simulink model "comm8qamtxrxhdl"  (R2025b)
settings: Solver=FixedStepDiscrete  StartTime=0.0  StopTime=20000*qam_params.symbolPeriod  RelTol=1e-3
PreLoadFcn:
  | qam_params = comm8qamtxrxhdl_init;
InitFcn:
  | qam_params = comm8qamtxrxhdl_init;
StopFcn:
  | comm8qamtxrxhdl_analyze;
undefined symbols (not defined in the file or in its folder): Add, Shift
libraries: hdlsllib x5, dspsigops x2, dspmlti4 x2, commchan3 x1, commrflib2 x1, simulink x1, dsphdlmathfun2 x1, dsphdlsigops2 x1, simulink_need_slupdate x1, commdigbbndam3 x1, commsequence2 x1
settings Model: Creator=The MathWorks, Inc.  LastModifiedBy=Ubaid
settings SolverCC: AlgebraicLoopSolver=TrustRegion  MaxZcPerStep=1.0
settings DataIOCC: LimitDataPoints=on  SaveFormat=Array  SaveOutput=off  SaveTime=off  ReturnWorkspaceOutputs=off
settings OptimizationCC: BlockReduction=off  ConditionallyExecuteInputs=off  DefaultParameterBehavior=Inlined  ReuseModelBlockBuffer=off  LifeSpan=inf
settings DebuggingCC: AlgebraicLoopMsg=error  UnderspecifiedInitializationDetection=Classic  MergeDetectMultiDrivingBlocksExec=none  SolverPrmCheckMsg=warning  MultiTaskDSMMsg=warning  MultiTaskCondExecSysMsg=none  SingleTaskRateTransMsg=error  IntegerOverflowMsg=none  ParameterPrecisionLossMsg=none  UnconnectedInputMsg=warning  UnconnectedOutputMsg=warning  UnconnectedLineMsg=warning  AllowSymbolicDim=off  StateNameClashWarn=warning  SFUnexpectedBacktrackingDiag=warning  SFNoUnconditionalDefaultTransitionDiag=warning  SFExecutionAtInitializationDiag=none  IntegerSaturationMsg=none  ArithmeticOperatorsInVariantConditions=warning
settings HardwareCC: ProdBitPerPointer=32.0  ProdBitPerSizeT=32.0  ProdBitPerPtrDiffT=32.0  ProdLargestAtomicFloat=None  ProdIntDivRoundTo=Undefined  ProdEndianess=Unspecified  ProdWordSize=32.0  ProdHWDeviceType=ASIC/FPGA->ASIC/FPGA  ProdEqTarget=off
settings ModelReferenceCC: EnableRefExpFcnMdlSchedulingChecks=on  PropagateSignalLabelsOutOfModel=off
settings SFSimCC: SimUseLocalCustomCode=off  CustomCodeUndefinedFunction=UseInterfaceOnly
settings RTWCC: RTWUseLocalCustomCode=off  GPUComputeCapability=3.5  DLArmComputeVersion=19.05
settings CodeAppCC: StateflowObjectComments=on
settings GRTTargetCC: TargetLangStandard=C89/C90 (ANSI)
settings ConfigComp: CovMetricSettings=dw  CovSaveCumulativeToWorkspaceVar=on  CovSaveSingleToWorkspaceVar=on  CovExternalEMLEnable=off  CovSFcnEnable=off

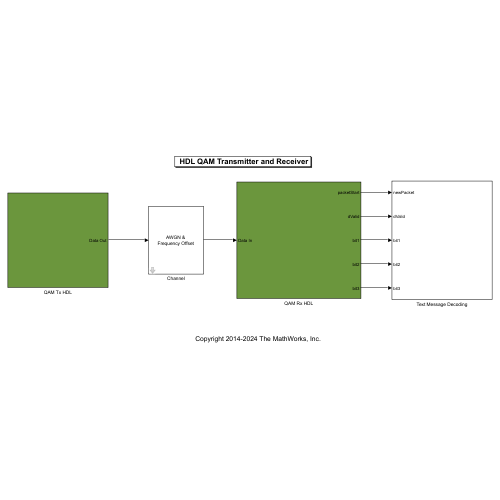
[thumbnail: Simulink's stored preview of the top-level diagram]
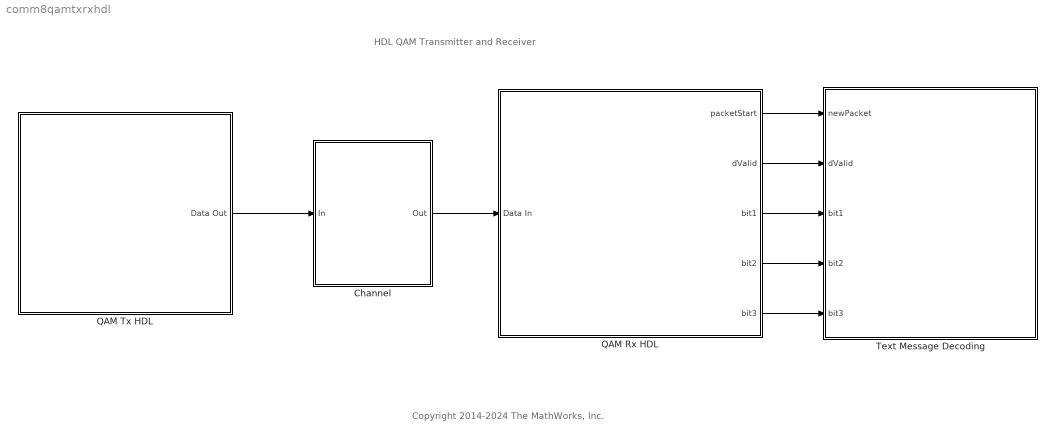
== system comm8qamtxrxhdl ==
  note: Copyright 2014-2024 The MathWorks, Inc.
  note: HDL QAM Transmitter and Receiver
  Channel : Subsystem  mask{Poff=qam_params.phaseOffset, Foff=qam_params.frequencyOffset, EbNo=qam_params.EbNo, Chan_Gain=qam_params.channelGain, Chan_Delay=qam_params.channelDelay}
      mask prompts: Poff "Phase offset (deg)"; Foff "Frequency offset (Hz)"; EbNo "Eb/No"; Chan_Gain "Channel Gain"; Chan_Delay "Channel Delay"
      mask Display: disp('AWGN &\nFrequency Offset');
  QAM Rx HDL : Subsystem
  QAM Tx HDL : Subsystem
  Text Message Decoding : Subsystem
  wires:
  QAM Rx HDL/1(packetStart) -> Text Message Decoding/1(newPacket)
  QAM Rx HDL/3(bit1) -> Text Message Decoding/3(bit1)
  QAM Rx HDL/4(bit2) -> Text Message Decoding/4(bit2)
  QAM Rx HDL/5(bit3) -> Text Message Decoding/5(bit3)
  QAM Rx HDL/2(dValid) -> Text Message Decoding/2(dValid)
  Channel/1(Out) -> QAM Rx HDL/1(Data In)
  QAM Tx HDL/1(Data Out) -> Channel/1(In)

== system comm8qamtxrxhdl/Channel ==
  In : Inport
  AWGN Channel2 : commchan3/AWGN Channel  LegacyMode=on  NoiseMethod="Signal to noise ratio  (Eb/No)"  noiseMode="Signal to noise ratio  (SNR)"  EbNo=EbNo  EsNo=15  SNR=15  BitsPerSymbol=3  SignalPower=0.11  SpecifySymbolPeriod=off  SamplesPerSymbol=1  SymbolPeriod=1/qam_params.sampleRate  VarianceSource=Parameter  Variance=1  RandomStream=Global stream  Seed=67  SimulateUsing=Code generation
  Constant : Constant  Value=Chan_Delay  SampleTime=1/qam_params.sampleRate
  Data Type Conversion1 : DataTypeConversion  OutDataTypeStr=fixdt(1,16,15)  SaturateOnIntegerOverflow=off  RndMeth=Floor
  Data Type Conversion4 : DataTypeConversion  OutDataTypeStr=double  SaturateOnIntegerOverflow=off  RndMeth=Floor
  Gain : Gain  Gain=Chan_Gain
  Phase/ Frequency Offset1 : commrflib2/Phase// Frequency Offset  phaseOffset=Poff  freqPort=off  freqOffset=Foff
  Variable Fractional Delay : dspsigops/Variable Fractional Delay  mode=OBSOLETE  modeActive=Linear  L=4  FarrowL=4  R=10  alpha=1  dmax=56*4  ic=0  noDFT=off  fallbackFIR=Clip to the minimum value necessary for centered kernel  fallbackFarrow=Clip to the minimum value necessary for centered kernel  roundingMode=Zero  overflowMode=off
  Out : Outport  VectorParamsAs1DForOutWhenUnconnected=off
  wires:
  In/1 -> Data Type Conversion4/1
  AWGN Channel2/1 -> Gain/1
  Data Type Conversion1/1 -> Out/1
  Data Type Conversion4/1 -> Phase/ Frequency Offset1/1
  Phase/ Frequency Offset1/1 -> Variable Fractional Delay/1
  Variable Fractional Delay/1 -> AWGN Channel2/1
  Constant/1 -> Variable Fractional Delay/2
  Gain/1 -> Data Type Conversion1/1

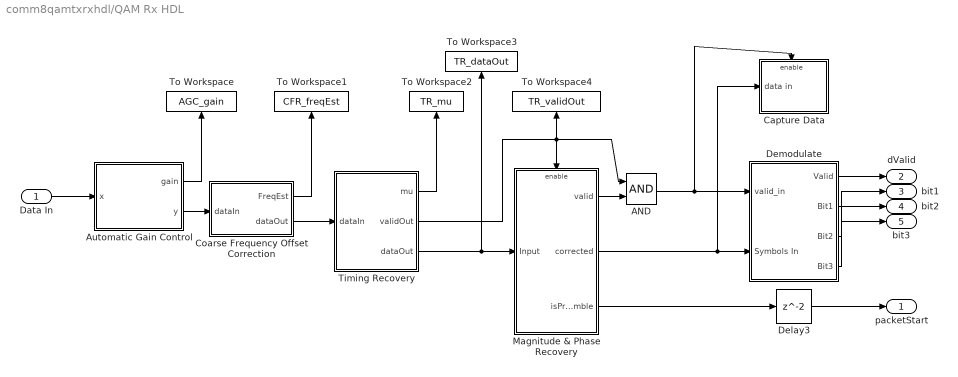
== system comm8qamtxrxhdl/QAM Rx HDL ==
  Data In : Inport
  AND : Logic  AllPortsSameDT=off  OutDataTypeStr=boolean
  Automatic Gain Control : Subsystem  mask{AGC_Ref=.23, AGC_Gain=0.001}
      mask prompts: AGC_Ref "Target Amplitude"; AGC_Gain "AGC Loop Gain"
  Capture Data : Subsystem
  Coarse Frequency Offset Correction : Subsystem
  Delay3 : Delay  InitialCondition=0
  Demodulate : Subsystem
  Magnitude & Phase Recovery : Subsystem  mask{PreAmb=qam_params.preambleRx.', threshold=1.1, LMS_Step=1/4}
      mask prompts: PreAmb "Preamble symbols"; LMS_Step "LMS step size"
  Timing Recovery : Subsystem
  To Workspace : ToWorkspace  VariableName=AGC_gain  SaveFormat=Timeseries  SampleTime=-1
  To Workspace1 : ToWorkspace  VariableName=CFR_freqEst  SaveFormat=Timeseries  SampleTime=-1
  To Workspace2 : ToWorkspace  VariableName=TR_mu  SaveFormat=Timeseries  SampleTime=-1
  To Workspace3 : ToWorkspace  VariableName=TR_dataOut  SaveFormat=Timeseries  SampleTime=-1
  To Workspace4 : ToWorkspace  VariableName=TR_validOut  SaveFormat=Timeseries  SampleTime=-1
  packetStart : Outport  VectorParamsAs1DForOutWhenUnconnected=off
  dValid : Outport  Port=2  VectorParamsAs1DForOutWhenUnconnected=off
  bit1 : Outport  Port=3  VectorParamsAs1DForOutWhenUnconnected=off
  bit2 : Outport  Port=4  VectorParamsAs1DForOutWhenUnconnected=off
  bit3 : Outport  Port=5  VectorParamsAs1DForOutWhenUnconnected=off
  wires:
  Timing Recovery/3(dataOut) -> Magnitude & Phase Recovery/1(Input), To Workspace3/1
  Demodulate/2(Bit1) -> bit1/1
  Demodulate/3(Bit2) -> bit2/1
  Demodulate/4(Bit3) -> bit3/1
  Magnitude & Phase Recovery/3(isPreamble) -> Delay3/1
  Demodulate/1(Valid) -> dValid/1
  Timing Recovery/2(validOut) -> AND/1, To Workspace4/1, Magnitude & Phase Recovery/Enable
  Data In/1 -> Automatic Gain Control/1(x)
  Automatic Gain Control/1(gain) -> To Workspace/1
  Automatic Gain Control/2(y) -> Coarse Frequency Offset Correction/1(dataIn)
  Coarse Frequency Offset Correction/2(dataOut) -> Timing Recovery/1(dataIn)
  Delay3/1 -> packetStart/1
  Magnitude & Phase Recovery/1(valid) -> AND/2
  AND/1 -> Demodulate/1(valid_in), Capture Data/Enable
  Magnitude & Phase Recovery/2(corrected) -> Demodulate/2(Symbols In), Capture Data/1(data in)
  Coarse Frequency Offset Correction/1(FreqEst) -> To Workspace1/1
  Timing Recovery/1(mu) -> To Workspace2/1

== system comm8qamtxrxhdl/QAM Tx HDL ==
  " Zero" : Constant  Value=complex(0,0)  OutDataTypeStr=fixdt(1,16,15)  SampleTime=qam_params.symbolPeriod
  Data Generation & Packetization : Subsystem
  Input Mux : MultiPortSwitch  DataPortOrder=Zero-based contiguous  Inputs=2  zeroidx=on  SaturateOnIntegerOverflow=off  InputSameDT=off
  Pipeline{1..5} (5 alike) : Delay  DelayLength=1  InitialCondition=0
  Pulse Shaping : Subsystem
  Symbol Mapping : Subsystem
  Data Out : Outport  VectorParamsAs1DForOutWhenUnconnected=off
  wires:
  Pipeline4/1 -> Input Mux/3
  Pipeline5/1 -> Data Out/1
  Pipeline1/1 -> Symbol Mapping/1(Valid In)
  Pipeline3/1 -> Input Mux/1
  " Zero"/1 -> Input Mux/2
  Data Generation & Packetization/1(Valid Out) -> Pipeline1/1
  Data Generation & Packetization/2(Raw Data) -> Pipeline2/1
  Pipeline2/1 -> Symbol Mapping/2(Integer In)
  Symbol Mapping/2(Symbol Out) -> Pipeline4/1
  Symbol Mapping/1(Valid out) -> Pipeline3/1
  Input Mux/1 -> Pulse Shaping/1(dataIn)
  Pulse Shaping/1(dataOut) -> Pipeline5/1

== system comm8qamtxrxhdl/Text Message Decoding ==
  newPacket : Inport
  dValid : Inport  Port=2
  bit1 : Inport  Port=3
  bit2 : Inport  Port=4
  bit3 : Inport  Port=5
  " " : MATLAB Function  TreatAsAtomicUnit=on
  Descramble and Print : Subsystem  TreatAsAtomicUnit=on
  wires:
  bit1/1 -> " "/3(bit1)
  bit2/1 -> " "/4(bit2)
  " "/2(framed_data) -> Descramble and Print/1(In1)
  " "/1(RxGo) -> Descramble and Print/Enable
  bit3/1 -> " "/5(bit3)
  dValid/1 -> " "/2(dValid)
  newPacket/1 -> " "/1(newPacket)

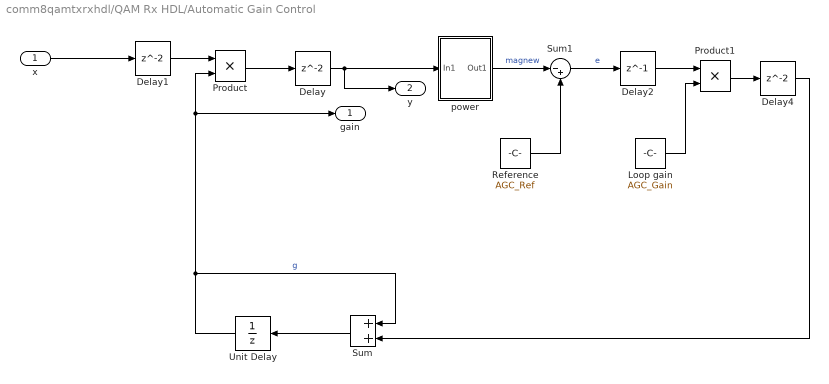
== system comm8qamtxrxhdl/QAM Rx HDL/Automatic Gain Control ==
  x : Inport
  Delay : Delay  InitialCondition=0
  Delay1 : Delay  InitialCondition=0
  Delay2 : Delay  DelayLength=1  InitialCondition=0
  Delay4 : Delay  InitialCondition=0
  Loop gain : Constant  Value=AGC_Gain  OutDataTypeStr=fixdt(1,16,15)  SampleTime=1/qam_params.sampleRate
  Product : Product  OutDataTypeStr=fixdt(1,16,15)  SaturateOnIntegerOverflow=on
  Product1 : Product  OutDataTypeStr=fixdt(1,16,15)  SaturateOnIntegerOverflow=on
  Reference : Constant  Value=AGC_Ref  OutDataTypeStr=fixdt(1,16,15)  SampleTime=1/qam_params.sampleRate
  Sum : Sum  OutDataTypeStr=Inherit: Same as accumulator  AccumDataTypeStr=fixdt(1,24,15)  SaturateOnIntegerOverflow=on
  Sum1 : Sum  Inputs=|-+  OutDataTypeStr=Inherit: Same as first input
  Unit Delay : UnitDelay  InitialCondition=.5  SampleTime=-1  HasFrameUpgradeWarning=on
  power : Subsystem
  gain : Outport  VectorParamsAs1DForOutWhenUnconnected=off
  y : Outport  Port=2  PortDimensions=1  VectorParamsAs1DForOutWhenUnconnected=off
  wires:
  Product/1 -> Delay/1
  Delay/1 -> y/1, power/1(In1)
  Sum1/1 -> Delay2/1  "e"
  Delay2/1 -> Product1/1
  Product1/1 -> Delay4/1
  Unit Delay/1 -> gain/1, Product/2, Sum/1  "g"
  Delay4/1 -> Sum/2
  x/1 -> Delay1/1
  Loop gain/1 -> Product1/2
  Sum/1 -> Unit Delay/1
  Reference/1 -> Sum1/2
  power/1(Out1) -> Sum1/1  "magnew"
  Delay1/1 -> Product/1

== system comm8qamtxrxhdl/QAM Rx HDL/Capture Data ==
  data in : Inport
  Enable : EnablePort
  To Workspace2 : ToWorkspace  VariableName=symbolEstimates  SaveFormat=Timeseries  SampleTime=-1
  wires:
  data in/1 -> To Workspace2/1

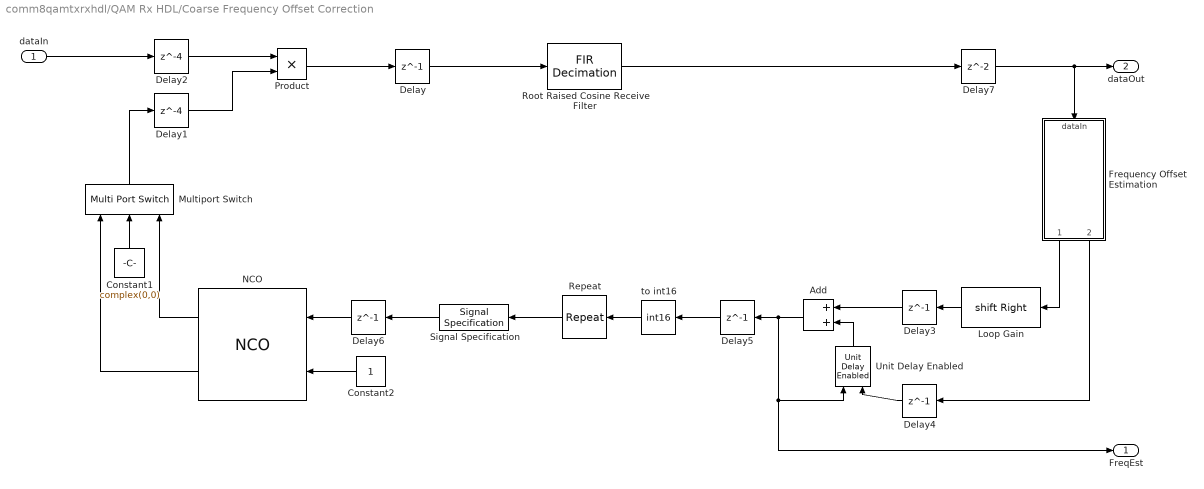
== system comm8qamtxrxhdl/QAM Rx HDL/Coarse Frequency Offset Correction ==
  dataIn : Inport
  Add : Sum  AccumDataTypeStr=fixdt(1,16,3)
  Constant1 : Constant  Value=complex(0,0)  OutDataTypeStr=fixdt(1,16,15)  SampleTime=1/qam_params.sampleRate
  Constant2 : Constant  OutDataTypeStr=boolean  SampleTime=1/qam_params.sampleRate
  Delay{,3..6} (5 alike) : Delay  DelayLength=1  InitialCondition=0
  Delay1 : Delay  DelayLength=4  InitialCondition=0
  Delay2 : Delay  DelayLength=4  InitialCondition=0
  Delay7 : Delay  InitialCondition=0
  Frequency Offset Estimation : Subsystem  mask{M=64, N=256, avFilterCoeffs=0}
      mask prompts: M "M (Luise Parameter)"; N "N (Luise Parameter)"; avFilterCoeffs "Filter Coeffs"
      mask init:
      | avFilterCoeffs = 1./(N*ones(1,M));
  Loop Gain : ArithShift  BinPtShiftNumber=-3  BitShiftDirection=Right
  Multiport Switch : MultiPortSwitch  DataPortOrder=Zero-based contiguous  Inputs=2  zeroidx=on  SaturateOnIntegerOverflow=off  InputSameDT=off
  NCO : dsphdlsigops2/NCO  PhaseIncrementSource=Input port  PhaseIncrement=100  PhaseOffsetSource=Property  PhaseOffset=0  DitherSource=Property  NumDitherBits=4  SamplesPerFrame=1  LUTCompress=off  ResetAction=off  Waveform=Complex exponential  PhasePort=off  SimulateUsing=Code generation  AccumulatorWL=16  PhaseQuantization=on  NumQuantizerAccumulatorBits=16  OutputDataType=Binary point scaling  OutputWL=16  OutputFL=15
  Product : Product  OutDataTypeStr=fixdt(1,16,15)
  Repeat : dspsigops/Repeat  FactorSource=Dialog parameter  N=2  Nmax=16  InputProcessing=Columns as channels (frame based)  RateOptions=Allow multirate processing  ic=0  mode=Unused parameter value
  Root Raised Cosine Receive Filter : dspmlti4/FIR Decimation  FilterSource=Dialog parameters  h=qam_params.ReceiverFilterCoefficients  D=2  filtStruct=Direct form transposed  FilterObject=Hm_firdecim  framing=Allow multirate processing  AllowArbitraryInputLength=off  inputOffset=0  outputBufInitCond=0  roundingMode=Floor  overflowMode=off  firstCoeffDataTypeStr=Inherit: Same word length as input  firstCoeffMin=[]  firstCoeffMax=[]  firstCoeffLastDataTypeStr=Inherit: Same word length as input  prodOutputMode=Binary point scaling  prodOutputWordLength=16  prodOutputFracLength=15  prodOutputDataTypeStr=fixdt(1,16,15)  prodOutputLastDataTypeStr=fixdt(1,16,15)  accumMode=Binary point scaling  accumWordLength=16  accumFracLength=15  accumDataTypeStr=fixdt(1,16,15)  accumLastDataTypeStr=fixdt(1,16,15)  outputMode=Binary point scaling  outputWordLength=16  outputFracLength=15  outputDataTypeStr=fixdt(1,16,15)  outputMin=[]  outputMax=[]  outputLastDataTypeStr=fixdt(1,16,15)
  Signal Specification : SignalSpecification  OutDataTypeStr=int16  Dimensions=1
  Unit Delay Enabled : simulink_need_slupdate/Unit Delay Enabled  vinit=0.0  tsamp=-1
  to int16 : DataTypeConversion  OutDataTypeStr=int16  SaturateOnIntegerOverflow=off  RndMeth=Floor
  FreqEst : Outport  VectorParamsAs1DForOutWhenUnconnected=off
  dataOut : Outport  Port=2  VectorParamsAs1DForOutWhenUnconnected=off
  wires:
  Product/1 -> Delay/1
  dataIn/1 -> Delay2/1
  Root Raised Cosine Receive Filter/1 -> Delay7/1
  Loop Gain/1 -> Delay3/1
  Frequency Offset Estimation/2(Estimate Valid) -> Delay4/1
  Constant2/1 -> NCO/2
  Signal Specification/1 -> Delay6/1
  Frequency Offset Estimation/1(Estimate) -> Loop Gain/1
  Repeat/1 -> Signal Specification/1
  to int16/1 -> Repeat/1
  Add/1 -> FreqEst/1, Unit Delay Enabled/1, Delay5/1
  Delay/1 -> Root Raised Cosine Receive Filter/1
  Delay1/1 -> Product/2
  Delay2/1 -> Product/1
  Delay3/1 -> Add/1
  Delay4/1 -> Unit Delay Enabled/2
  Unit Delay Enabled/1 -> Add/2
  Delay7/1 -> dataOut/1, Frequency Offset Estimation/1(dataIn)
  Delay6/1 -> NCO/1
  NCO/1 -> Multiport Switch/3
  NCO/2 -> Multiport Switch/1
  Multiport Switch/1 -> Delay1/1
  Constant1/1 -> Multiport Switch/2
  Delay5/1 -> to int16/1

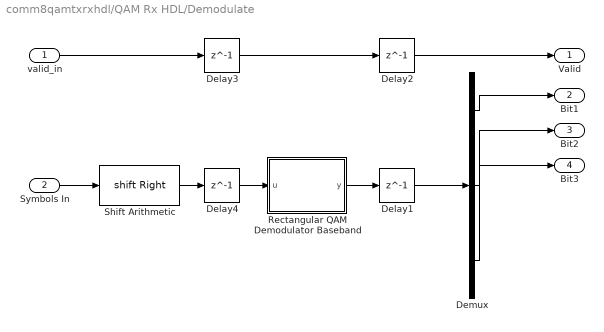
== system comm8qamtxrxhdl/QAM Rx HDL/Demodulate ==
  valid_in : Inport
  Symbols In : Inport  Port=2
  Delay{1..4} (4 alike) : Delay  DelayLength=1  InitialCondition=0
  Demux : Demux  Outputs=3
  Rectangular QAM Demodulator Baseband : MATLAB Function  TreatAsAtomicUnit=on
  Shift Arithmetic : ArithShift  BinPtShiftNumber=2  BitShiftDirection=Right
  Valid : Outport  VectorParamsAs1DForOutWhenUnconnected=off
  Bit1 : Outport  Port=2  VectorParamsAs1DForOutWhenUnconnected=off
  Bit2 : Outport  Port=3  VectorParamsAs1DForOutWhenUnconnected=off
  Bit3 : Outport  Port=4  VectorParamsAs1DForOutWhenUnconnected=off
  wires:
  Demux/1 -> Bit1/1
  valid_in/1 -> Delay3/1
  Demux/2 -> Bit2/1
  Demux/3 -> Bit3/1
  Symbols In/1 -> Shift Arithmetic/1
  Shift Arithmetic/1 -> Delay4/1
  Delay1/1 -> Demux/1
  Delay2/1 -> Valid/1
  Delay3/1 -> Delay2/1
  Delay4/1 -> Rectangular QAM Demodulator Baseband/1(u)
  Rectangular QAM Demodulator Baseband/1(y) -> Delay1/1

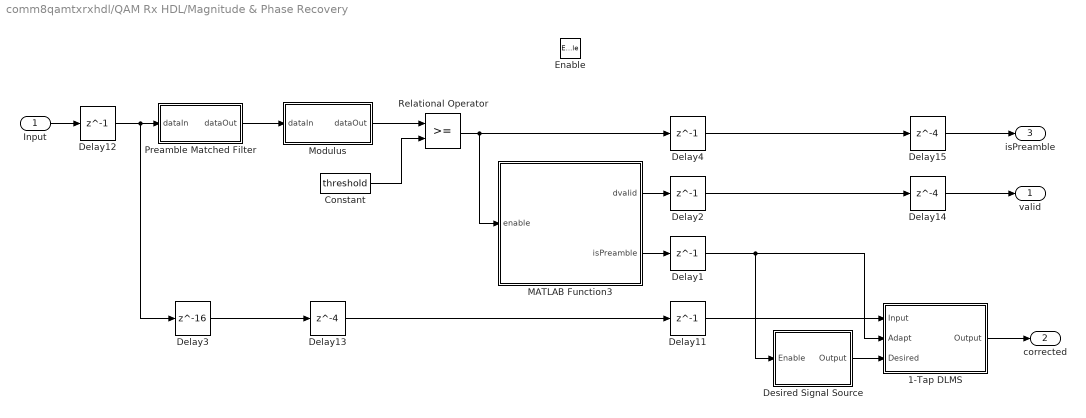
== system comm8qamtxrxhdl/QAM Rx HDL/Magnitude & Phase Recovery ==
  Input : Inport
  Enable : EnablePort
  1-Tap DLMS : Subsystem
  Constant : Constant  Value=threshold  OutDataTypeStr=Inherit: Inherit via back propagation  SampleTime=1/(qam_params.sampleRate/2)
  Delay{1..2,4,11..12} (5 alike) : Delay  DelayLength=1  InitialCondition=0
  Delay13 : Delay  DelayLength=4  InitialCondition=0
  Delay14 : Delay  DelayLength=4  InitialCondition=0
  Delay15 : Delay  DelayLength=4  InitialCondition=0
  Delay3 : Delay  DelayLength=16  InitialCondition=0
  Desired Signal Source : Subsystem
  MATLAB Function3 : MATLAB Function  TreatAsAtomicUnit=on
  Modulus : Subsystem
  Preamble Matched Filter : Subsystem
  Relational Operator : RelationalOperator  OutDataTypeStr=boolean
  valid : Outport  InitialOutput=0  VectorParamsAs1DForOutWhenUnconnected=off
  corrected : Outport  Port=2  InitialOutput=0  VectorParamsAs1DForOutWhenUnconnected=off
  isPreamble : Outport  Port=3  InitialOutput=0  VectorParamsAs1DForOutWhenUnconnected=off
  wires:
  MATLAB Function3/1(dvalid) -> Delay2/1
  MATLAB Function3/2(isPreamble) -> Delay1/1
  Modulus/1(dataOut) -> Relational Operator/1
  Relational Operator/1 -> MATLAB Function3/1(enable), Delay4/1
  Constant/1 -> Relational Operator/2
  Preamble Matched Filter/1(dataOut) -> Modulus/1(dataIn)
  Input/1 -> Delay12/1
  Delay3/1 -> Delay13/1
  Delay14/1 -> valid/1
  Delay15/1 -> isPreamble/1
  Delay2/1 -> Delay14/1
  Delay4/1 -> Delay15/1
  Delay12/1 -> Delay3/1, Preamble Matched Filter/1(dataIn)
  Delay11/1 -> 1-Tap DLMS/1(Input)
  Delay13/1 -> Delay11/1
  1-Tap DLMS/1(Output) -> corrected/1
  Delay1/1 -> 1-Tap DLMS/2(Adapt), Desired Signal Source/1(Enable)
  Desired Signal Source/1(Output) -> 1-Tap DLMS/3(Desired)

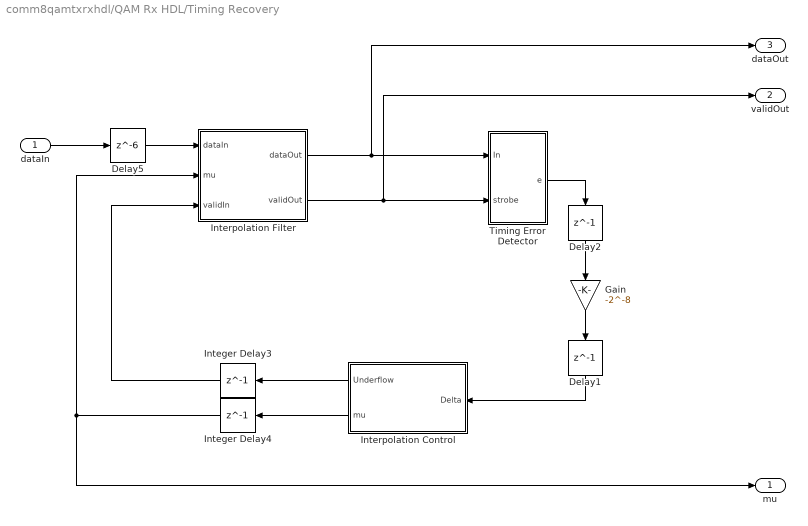
== system comm8qamtxrxhdl/QAM Rx HDL/Timing Recovery ==
  dataIn : Inport
  Delay1 : Delay  DelayLength=1
  Delay2 : Delay  DelayLength=1
  Delay5 : Delay  DelayLength=6
  Gain : Gain  Gain=-2^-8  OutDataTypeStr=fixdt(1,16,15)
  Integer Delay3 : Delay  DelayLength=1
  Integer Delay4 : Delay  DelayLength=1
  Interpolation Control : MATLAB Function
  "Interpolation Filter " : Subsystem
  Timing Error Detector : MATLAB Function  TreatAsAtomicUnit=on
  mu : Outport  VectorParamsAs1DForOutWhenUnconnected=off
  validOut : Outport  Port=2  VectorParamsAs1DForOutWhenUnconnected=off
  dataOut : Outport  Port=3  VectorParamsAs1DForOutWhenUnconnected=off
  wires:
  Interpolation Control/2(mu) -> Integer Delay4/1
  Interpolation Control/1(Underflow) -> Integer Delay3/1
  Integer Delay3/1 -> "Interpolation Filter "/3(validIn)
  "Interpolation Filter "/2(validOut) -> Timing Error Detector/2(strobe), validOut/1
  Integer Delay4/1 -> mu/1, "Interpolation Filter "/2(mu)
  Gain/1 -> Delay1/1
  Timing Error Detector/1(e) -> Delay2/1
  "Interpolation Filter "/1(dataOut) -> Timing Error Detector/1(In), dataOut/1
  dataIn/1 -> Delay5/1
  Delay5/1 -> "Interpolation Filter "/1(dataIn)
  Delay1/1 -> Interpolation Control/1(Delta)
  Delay2/1 -> Gain/1

== system comm8qamtxrxhdl/QAM Tx HDL/Data Generation & Packetization ==
  Controller FSM : MATLAB Function  TreatAsAtomicUnit=on  SystemSampleTime=1/qam_params.bitRate
  Data Source : Subsystem
  Downsample : DownSample  N=3  RateOptions=Allow multirate processing
  Group Bits : Subsystem
  Pipeline : Delay  InitialCondition=0
  Pipeline1 : Delay  DelayLength=1  InitialCondition=0
  Pipeline2 : Delay  DelayLength=1  InitialCondition=0
  Valid : Constant  OutDataTypeStr=boolean  SampleTime=1/qam_params.bitRate
  Valid Out : Outport  VectorParamsAs1DForOutWhenUnconnected=off
  Raw Data : Outport  Port=2  VectorParamsAs1DForOutWhenUnconnected=off
  wires:
  Data Source/1(packet_bits) -> Pipeline2/1
  Valid/1 -> Pipeline/1
  Pipeline1/1 -> Downsample/1
  Pipeline/1 -> Pipeline1/1
  Downsample/1 -> Valid Out/1
  Pipeline2/1 -> Group Bits/1(Bits In)
  Group Bits/1(Integer Out) -> Raw Data/1
  Controller FSM/3(load_data) -> Data Source/3(load data)
  Controller FSM/2(load_preamble) -> Data Source/2(load preamble)
  Controller FSM/1(reset_preamble) -> Data Source/1(reset preamble)

== system comm8qamtxrxhdl/QAM Tx HDL/Pulse Shaping ==
  dataIn : Inport
  RRC Interpolation Filter : dspmlti4/FIR Interpolation  FilterSource=Dialog parameters  PrivateCoeffs=0  h=qam_params.TransmitterFilterCoefficients  L=4  FilterObject=Htxrc  framing=Allow multirate processing  outputBufInitCond=0  roundingMode=Nearest  overflowMode=on  firstCoeffMode=Binary point scaling  firstCoeffWordLength=16  firstCoeffFracLength=15  firstCoeffDataTypeStr=fixdt(1,16,15)  firstCoeffMin=[]  firstCoeffMax=[]  firstCoeffLastDataTypeStr=fixdt(1,16,15)  prodOutputMode=Binary point scaling  prodOutputWordLength=16  prodOutputFracLength=15  prodOutputDataTypeStr=fixdt(1,16,15)  prodOutputLastDataTypeStr=fixdt(1,16,15)  accumMode=Binary point scaling  accumWordLength=16  accumFracLength=15  accumDataTypeStr=fixdt(1,16,15)  accumLastDataTypeStr=fixdt(1,16,15)  outputMode=Binary point scaling  outputWordLength=16  outputFracLength=15  outputDataTypeStr=fixdt(1,16,15)  outputMin=[]  outputMax=[]  outputLastDataTypeStr=fixdt(1,16,15)
  dataOut : Outport  VectorParamsAs1DForOutWhenUnconnected=off
  wires:
  RRC Interpolation Filter/1 -> dataOut/1
  dataIn/1 -> RRC Interpolation Filter/1

== system comm8qamtxrxhdl/QAM Tx HDL/Symbol Mapping ==
  Valid In : Inport
  Integer In : Inport  Port=2
  Rectangular QAM Modulator Baseband : commdigbbndam3/Rectangular QAM Modulator Baseband  M=8  InType=Integer  Enc=Gray  Mapping=[0:15]  PowType=Min. distance between symbols  MinDist=0.5  AvgPow=.66  PeakPow=1.1  Ph=0  outDtype=Fixed-point  outWordLen=16  outUDDataType=sfix(16)  outFracLenMode=Best precision  outFracLen=15  outDataTypeStr=fixdt(1,16)  outLastDataTypeStr=fixdt(1,16)
  Valid out : Outport  VectorParamsAs1DForOutWhenUnconnected=off
  Symbol Out : Outport  Port=2  VectorParamsAs1DForOutWhenUnconnected=off
  wires:
  Rectangular QAM Modulator Baseband/1 -> Symbol Out/1
  Integer In/1 -> Rectangular QAM Modulator Baseband/1
  Valid In/1 -> Valid out/1

== system comm8qamtxrxhdl/Text Message Decoding/Descramble and Print ==
  In1 : Inport
  Enable : EnablePort
  BitsToDecimal1 : MATLAB Function  TreatAsAtomicUnit=on
  Descrambler : commsequence2/Descrambler  M=2  poly=[1 1 1 0 1]  iniStaSource=Dialog Parameter  ini_sta=[0 0 0 0]  resetViaPort=off
  Selector : Selector  IndexOptions=Index vector (dialog)  Indices=[43:1:168]  OutputSizes=1
  Selector1 : Selector  IndexOptions=Index vector (dialog)  Indices=[1:1:126]  OutputSizes=1
  wires:
  Selector1/1 -> BitsToDecimal1/1(u)
  In1/1 -> Selector/1
  Selector/1 -> Descrambler/1
  Descrambler/1 -> Selector1/1

== system comm8qamtxrxhdl/QAM Rx HDL/Automatic Gain Control/power ==
  In1 : Inport
  Complex to Real-Imag : ComplexToRealImag
  Delay : Delay  InitialCondition=0
  Delay1 : Delay  InitialCondition=0
  Delay2 : Delay  InitialCondition=0
  Product3 : Product  OutDataTypeStr=fixdt(1,16,15)  SaturateOnIntegerOverflow=on
  Product4 : Product  OutDataTypeStr=fixdt(1,16,15)  SaturateOnIntegerOverflow=on
  Sum1 : Sum  OutDataTypeStr=fixdt(1,16,14)  AccumDataTypeStr=fixdt(1,16,15)  SaturateOnIntegerOverflow=on
  Out1 : Outport  VectorParamsAs1DForOutWhenUnconnected=off
  wires:
  Product3/1 -> Delay/1
  Complex to Real-Imag/1 -> Product3/2, Product3/1
  Complex to Real-Imag/2 -> Product4/1, Product4/2
  Product4/1 -> Delay1/1
  Sum1/1 -> Delay2/1
  Delay/1 -> Sum1/1
  Delay1/1 -> Sum1/2
  In1/1 -> Complex to Real-Imag/1
  Delay2/1 -> Out1/1

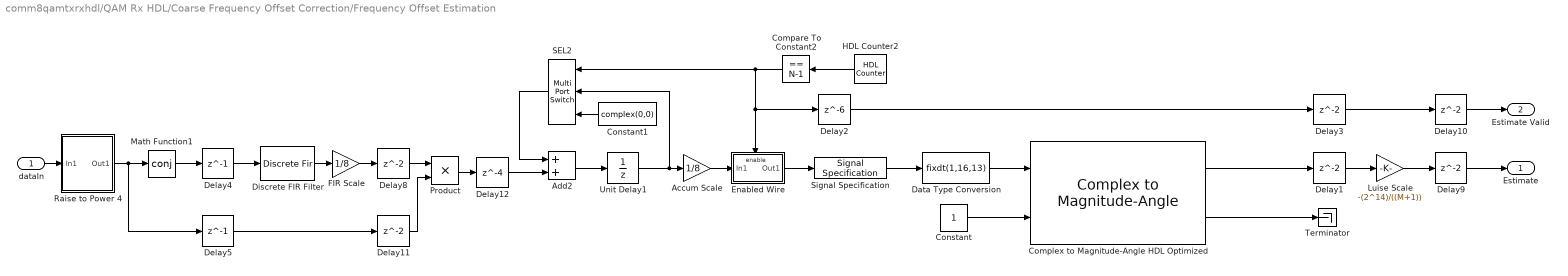
== system comm8qamtxrxhdl/QAM Rx HDL/Coarse Frequency Offset Correction/Frequency Offset Estimation ==
  dataIn : Inport
  Accum Scale : Gain  Gain=1/8  OutDataTypeStr=fixdt(1,32,31)
  Add2 : Sum  OutDataTypeStr=fixdt(1,32,28)
  Compare To Constant2 : simulink/Logic and Bit Operations/Compare To Constant  relop===  const=N-1  OutDataTypeStr=boolean
  Complex to Magnitude-Angle HDL Optimized : dsphdlmathfun2/Complex to Magnitude-Angle  NumIterationsSource=Property  NumIterations=5  OutputFormat=Angle  AngleFormat=Normalized  ScaleOutput=on  ScalingMethod=Shift-Add  SimulateUsing=Code generation
  Constant : Constant  OutDataTypeStr=boolean  SampleTime=5e-7
  Constant1 : Constant  Value=complex(0,0)  OutDataTypeStr=fixdt(1,32,28)  SampleTime=1/(qam_params.sampleRate/2)
  Data Type Conversion : DataTypeConversion  OutDataTypeStr=fixdt(1,16,13)  SaturateOnIntegerOverflow=off  RndMeth=Floor
  Delay{1,3,8..11} (6 alike) : Delay  InitialCondition=0
  Delay12 : Delay  DelayLength=4  InitialCondition=0
  Delay2 : Delay  DelayLength=6  InitialCondition=0
  Delay4 : Delay  DelayLength=1  InitialCondition=0
  Delay5 : Delay  DelayLength=1  InitialCondition=0
  Discrete FIR Filter : DiscreteFir  FilterStructure=Direct form transposed  Coefficients=ones(1,M)  CoefDataTypeStr=fixdt(1,2,0)  ProductDataTypeStr=fixdt(1,16,15)  AccumDataTypeStr=fixdt(1,19,15)  OutDataTypeStr=fixdt(1,19,15)
  Enabled Wire : Subsystem  TreatAsAtomicUnit=on
  FIR Scale : Gain  Gain=1/8  OutDataTypeStr=fixdt(1,19,18)
  HDL Counter2 : hdlsllib/Sources/HDL Counter  CountType=Count limited  CountInit=0  CountStep=1  CountMax=N-1  CountFromType=Initial value  CountFrom=0  CountResetPort=off  CountLoadPort=off  CountEnbPort=off  CountDirPort=off  CountHitOutputPort=off  CountDataType=Unsigned  CountWordLen=12  CountFracLen=0  CountSampTime=1/(qam_params.sampleRate/2)
  Luise Scale : Gain  Gain=-(2^14)/((M+1))  OutDataTypeStr=int16
  Math Function1 : Math  Operator=conj  SignedPower=on  OutputSignalType=complex
  Product : Product  OutDataTypeStr=fixdt(1,32,31)
  Raise to Power 4 : Subsystem
  SEL2 : MultiPortSwitch  DataPortOrder=Zero-based contiguous  Inputs=2  DiagnosticForDefault=None  zeroidx=on  OutDataTypeStr=fixdt(1,32,28)  SaturateOnIntegerOverflow=off  InputSameDT=off
  Signal Specification : SignalSpecification  Dimensions=1
  Terminator : Terminator
  Unit Delay1 : UnitDelay  InitialCondition=0+0j  SampleTime=-1  HasFrameUpgradeWarning=on
  Estimate : Outport  VectorParamsAs1DForOutWhenUnconnected=off
  Estimate Valid : Outport  Port=2  VectorParamsAs1DForOutWhenUnconnected=off
  wires:
  Delay9/1 -> Estimate/1
  Delay10/1 -> Estimate Valid/1
  dataIn/1 -> Raise to Power 4/1(In1)
  Delay2/1 -> Delay3/1
  Delay3/1 -> Delay10/1
  Complex to Magnitude-Angle HDL Optimized/1 -> Delay1/1
  Math Function1/1 -> Delay4/1
  Luise Scale/1 -> Delay9/1
  Enabled Wire/1(Out1) -> Signal Specification/1
  HDL Counter2/1 -> Compare To Constant2/1
  Raise to Power 4/1(Out1) -> Math Function1/1, Delay5/1
  Discrete FIR Filter/1 -> FIR Scale/1
  Delay11/1 -> Product/2
  Delay4/1 -> Discrete FIR Filter/1
  Delay5/1 -> Delay11/1
  FIR Scale/1 -> Delay8/1
  Delay8/1 -> Product/1
  Product/1 -> Delay12/1
  Constant1/1 -> SEL2/3
  Add2/1 -> Unit Delay1/1
  Unit Delay1/1 -> SEL2/2, Accum Scale/1
  SEL2/1 -> Add2/1
  Delay12/1 -> Add2/2
  Compare To Constant2/1 -> SEL2/1, Enabled Wire/Enable, Delay2/1
  Accum Scale/1 -> Enabled Wire/1(In1)
  Delay1/1 -> Luise Scale/1
  Constant/1 -> Complex to Magnitude-Angle HDL Optimized/2
  Complex to Magnitude-Angle HDL Optimized/2 -> Terminator/1
  Signal Specification/1 -> Data Type Conversion/1
  Data Type Conversion/1 -> Complex to Magnitude-Angle HDL Optimized/1

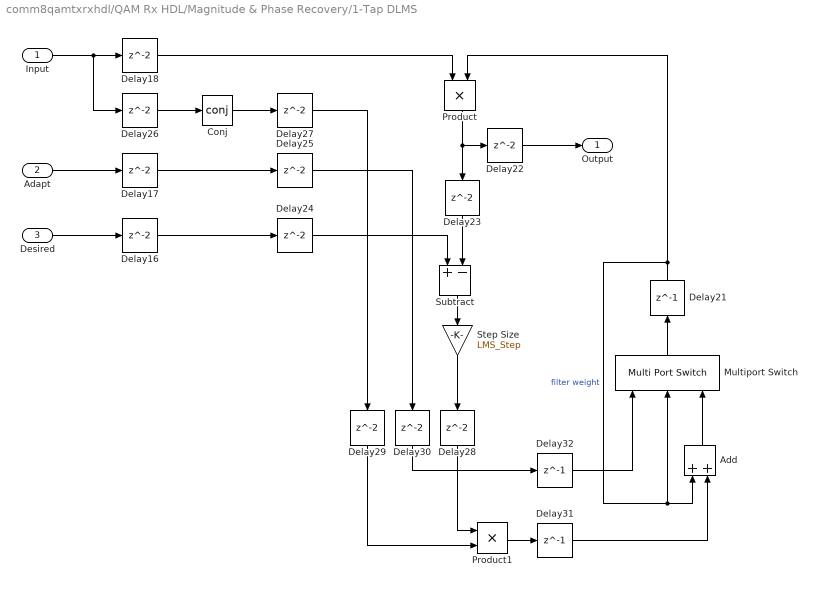
== system comm8qamtxrxhdl/QAM Rx HDL/Magnitude & Phase Recovery/1-Tap DLMS ==
  Input : Inport
  Adapt : Inport  Port=2
  Desired : Inport  Port=3
  Add : Sum  OutDataTypeStr=fixdt(1,17,14)
  Conj : Math  Operator=conj  SignedPower=on
  Delay{16..18,22..30} (12 alike) : Delay  InitialCondition=0
  Delay21 : Delay  DelayLength=1  InitialCondition=1
  Delay31 : Delay  DelayLength=1  InitialCondition=0
  Delay32 : Delay  DelayLength=1  InitialCondition=0
  Multiport Switch : MultiPortSwitch  DataPortOrder=Zero-based contiguous  Inputs=2  zeroidx=on  SaturateOnIntegerOverflow=off  InputSameDT=off
  Product : Product  OutDataTypeStr=fixdt(1,16,14)
  Product1 : Product  OutDataTypeStr=fixdt(1,16,15)
  Step Size : Gain  Gain=LMS_Step  OutDataTypeStr=fixdt(1,16,15)
  Subtract : Sum  Inputs=+-  AccumDataTypeStr=fixdt(1,16,14)
  Output : Outport  VectorParamsAs1DForOutWhenUnconnected=off
  wires:
  Adapt/1 -> Delay17/1
  Desired/1 -> Delay16/1
  Delay18/1 -> Product/1
  Delay16/1 -> Delay24/1
  Delay17/1 -> Delay25/1
  Add/1 -> Multiport Switch/3
  Delay21/1 -> Product/2, Multiport Switch/2, Add/1  "filter weight"
  Product/1 -> Delay23/1, Delay22/1
  Subtract/1 -> Step Size/1
  Multiport Switch/1 -> Delay21/1
  Input/1 -> Delay26/1, Delay18/1
  Delay23/1 -> Subtract/2
  Delay24/1 -> Subtract/1
  Delay26/1 -> Conj/1
  Delay22/1 -> Output/1
  Product1/1 -> Delay31/1
  Step Size/1 -> Delay28/1
  Delay27/1 -> Delay29/1
  Delay25/1 -> Delay30/1
  Delay28/1 -> Product1/1
  Delay29/1 -> Product1/2
  Delay30/1 -> Delay32/1
  Delay31/1 -> Add/2
  Delay32/1 -> Multiport Switch/1
  Conj/1 -> Delay27/1

== system comm8qamtxrxhdl/QAM Rx HDL/Magnitude & Phase Recovery/Desired Signal Source ==
  Enable : Inport
  HDL Counter2 : hdlsllib/Sources/HDL Counter  CountType=Count limited  CountInit=0  CountStep=1  CountMax=13  CountFromType=Initial value  CountFrom=0  CountResetPort=off  CountLoadPort=off  CountEnbPort=on  CountDirPort=off  CountHitOutputPort=off  CountDataType=Unsigned  CountWordLen=8  CountFracLen=0  CountSampTime=-1
  data lookup : LookupNDDirect  NumberOfTableDimensions=1  Table=PreAmb  DiagnosticForOutOfRangeInput=Error  TableDataTypeStr=fixdt(1,16,15)
  Output : Outport  VectorParamsAs1DForOutWhenUnconnected=off
  wires:
  Enable/1 -> HDL Counter2/1
  HDL Counter2/1 -> data lookup/1
  data lookup/1 -> Output/1

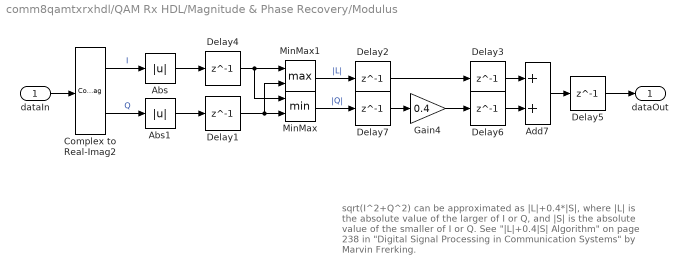
== system comm8qamtxrxhdl/QAM Rx HDL/Magnitude & Phase Recovery/Modulus ==
  note: sqrt(I^2+Q^2) can be approximated as |L|+0.4*|S|,
      | where |L| is the absolute value of the larger of I or Q,
      | and |S| is the absolute value of the smaller of I or Q.
      |
      | See "|L|+0.4|S| Algorithm" on page 238 in "Digital Signal
      | Processing in Communication Systems" by Marvin Frerking.
  dataIn : Inport
  Abs : Abs  SaturateOnIntegerOverflow=off
  Abs1 : Abs  SaturateOnIntegerOverflow=off
  Add7 : Sum
  Complex to Real-Imag2 : ComplexToRealImag
  Delay{1..7} (7 alike) : Delay  DelayLength=1  InitialCondition=0
  Gain4 : Gain  Gain=0.4  OutDataTypeStr=fixdt(1,16,15)
  MinMax : MinMax  Inputs=2
  MinMax1 : MinMax  Function=max  Inputs=2
  dataOut : Outport  VectorParamsAs1DForOutWhenUnconnected=off
  wires:
  dataIn/1 -> Complex to Real-Imag2/1
  Abs1/1 -> Delay1/1
  Abs/1 -> Delay4/1
  Gain4/1 -> Delay6/1
  MinMax1/1 -> Delay2/1  "|L|"
  MinMax/1 -> Delay7/1  "|Q|"
  Add7/1 -> Delay5/1
  Delay7/1 -> Gain4/1
  Delay2/1 -> Delay3/1
  Delay1/1 -> MinMax1/2, MinMax/2
  Delay4/1 -> MinMax1/1, MinMax/1
  Delay6/1 -> Add7/2
  Delay5/1 -> dataOut/1
  Delay3/1 -> Add7/1
  Complex to Real-Imag2/2 -> Abs1/1  "Q"
  Complex to Real-Imag2/1 -> Abs/1  "I"

== system comm8qamtxrxhdl/QAM Rx HDL/Magnitude & Phase Recovery/Preamble Matched Filter ==
  dataIn : Inport
  Add2 : Sum
  Add3 : Sum  Inputs=+-
  Complex to Real-Imag2 : ComplexToRealImag
  Delay{1..4} (4 alike) : Delay  DelayLength=1  InitialCondition=0
  Discrete FIR Filter3 : DiscreteFir  FilterStructure=Direct form transposed  Coefficients=real(fliplr(conj(PreAmb/7)))  CoefDataTypeStr=fixdt(1,16,15)  ProductDataTypeStr=fixdt(1,16,15)  AccumDataTypeStr=fixdt(1,17,15)  OutDataTypeStr=fixdt(1,17,15)
  Discrete FIR Filter4 : DiscreteFir  FilterStructure=Direct form transposed  Coefficients=-real(fliplr(conj(PreAmb/7)))  CoefDataTypeStr=fixdt(1,16,15)  ProductDataTypeStr=fixdt(1,16,15)  AccumDataTypeStr=fixdt(1,17,15)  OutDataTypeStr=fixdt(1,17,15)
  Real-Imag to Complex2 : RealImagToComplex
  dataOut : Outport  VectorParamsAs1DForOutWhenUnconnected=off
  wires:
  Delay1/1 -> Discrete FIR Filter4/1
  Delay3/1 -> Real-Imag to Complex2/2
  Delay2/1 -> Real-Imag to Complex2/1
  Delay4/1 -> Discrete FIR Filter3/1
  Add3/1 -> Delay1/1
  Discrete FIR Filter3/1 -> Delay2/1
  Add2/1 -> Delay4/1
  Discrete FIR Filter4/1 -> Delay3/1
  Complex to Real-Imag2/1 -> Add3/1, Add2/1
  Complex to Real-Imag2/2 -> Add2/2, Add3/2
  Real-Imag to Complex2/1 -> dataOut/1
  dataIn/1 -> Complex to Real-Imag2/1

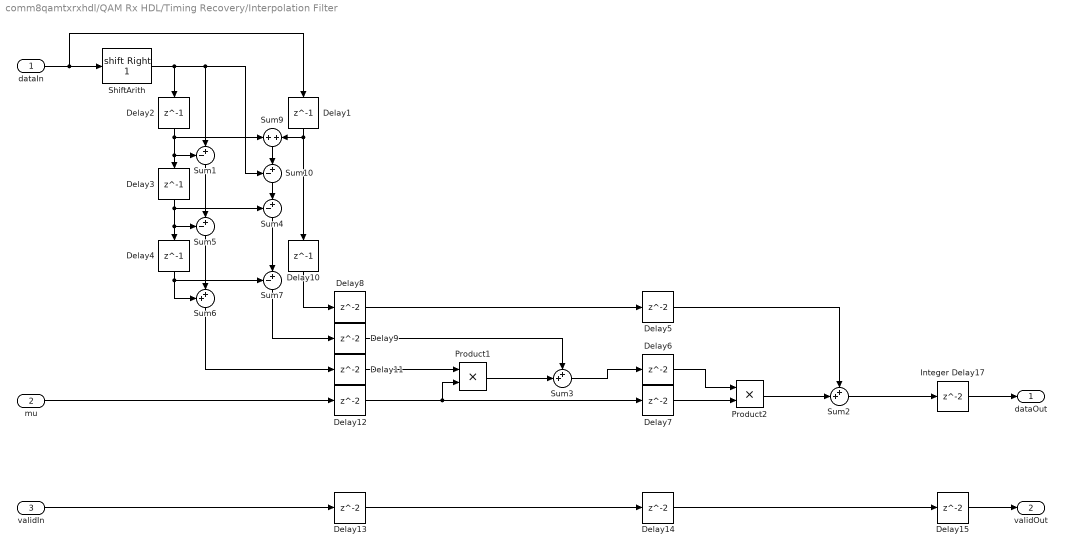
== system comm8qamtxrxhdl/QAM Rx HDL/Timing Recovery/Interpolation Filter  ==
  dataIn : Inport
  mu : Inport  Port=2
  validIn : Inport  Port=3
  Delay{1..4,10} (5 alike) : Delay  DelayLength=1  InitialCondition=0
  Delay{5..9,11..15} (10 alike) : Delay  InitialCondition=0
  Integer Delay17 : Delay  InitialCondition=0
  Product1 : Product  OutDataTypeStr=fixdt(1,16,14)  RndMeth=Zero
  Product2 : Product  OutDataTypeStr=fixdt(1,16,14)  RndMeth=Zero
  ShiftArith : ArithShift  BitShiftNumber=1  BitShiftDirection=Right
  Sum{1,4..5,7,10} (5 alike) : Sum  Inputs=-+|  OutDataTypeStr=fixdt(1,16,14)
  Sum2 : Sum  Inputs=++|  OutDataTypeStr=Inherit: Same as accumulator  AccumDataTypeStr=fixdt(1,16,15)
  Sum3 : Sum  Inputs=++|
  Sum6 : Sum  Inputs=++|  OutDataTypeStr=fixdt(1,16,14)  SaturateOnIntegerOverflow=on
  Sum9 : Sum  Inputs=+|+  OutDataTypeStr=fixdt(1,16,14)
  dataOut : Outport  VectorParamsAs1DForOutWhenUnconnected=off
  validOut : Outport  Port=2  VectorParamsAs1DForOutWhenUnconnected=off
  wires:
  ShiftArith/1 -> Sum10/1, Sum1/2, Delay2/1
  Delay1/1 -> Sum9/2, Delay10/1
  Delay2/1 -> Sum9/1, Delay3/1, Sum1/1
  Sum10/1 -> Sum4/2
  Delay3/1 -> Delay4/1, Sum5/1, Sum4/1
  Sum1/1 -> Sum5/2
  Delay4/1 -> Sum6/1, Sum7/1
  Sum5/1 -> Sum6/2
  Sum4/1 -> Sum7/2
  Delay6/1 -> Product2/1
  Sum3/1 -> Delay6/1
  Product2/1 -> Sum2/2
  Product1/1 -> Sum3/2
  Delay11/1 -> Product1/1
  Delay9/1 -> Sum3/1
  Delay8/1 -> Delay5/1
  Delay12/1 -> Delay7/1, Product1/2
  Delay7/1 -> Product2/2
  Delay5/1 -> Sum2/1
  Delay10/1 -> Delay8/1
  Sum7/1 -> Delay9/1
  mu/1 -> Delay12/1
  Integer Delay17/1 -> dataOut/1
  dataIn/1 -> Delay1/1, ShiftArith/1
  Sum2/1 -> Integer Delay17/1
  Sum9/1 -> Sum10/2
  validIn/1 -> Delay13/1
  Delay13/1 -> Delay14/1
  Delay14/1 -> Delay15/1
  Delay15/1 -> validOut/1
  Sum6/1 -> Delay11/1

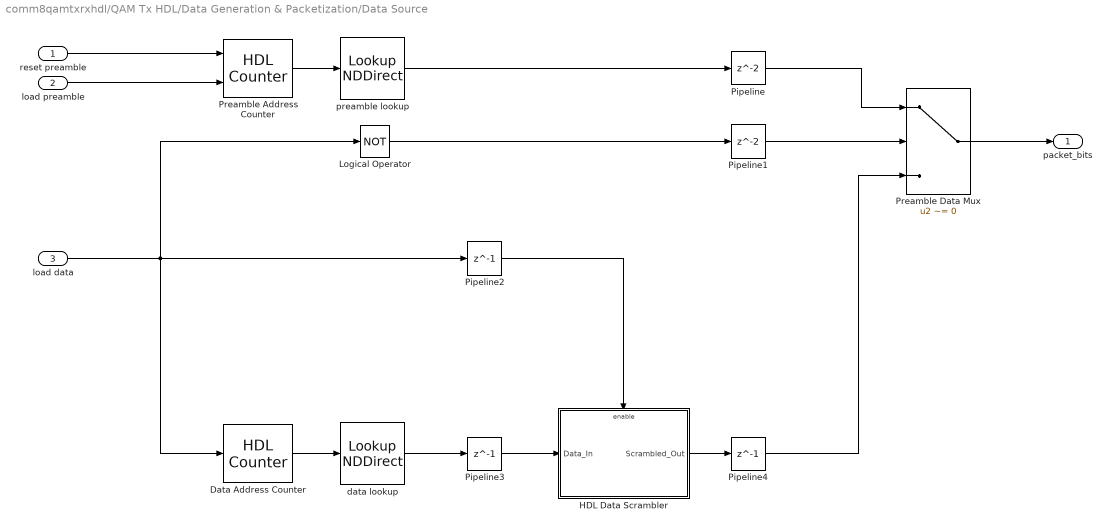
== system comm8qamtxrxhdl/QAM Tx HDL/Data Generation & Packetization/Data Source ==
  reset preamble : Inport
  load preamble : Inport  Port=2
  load data : Inport  Port=3
  Data Address Counter : hdlsllib/Sources/HDL Counter  CountType=Count limited  CountInit=0  CountStep=1  CountMax=qam_params.total_data_bits-1  CountFromType=Initial value  CountFrom=0  CountResetPort=off  CountLoadPort=off  CountEnbPort=on  CountDirPort=off  CountHitOutputPort=off  CountDataType=Unsigned  CountWordLen=16  CountFracLen=0  CountSampTime=1
  HDL Data Scrambler : Subsystem  TreatAsAtomicUnit=on
  Logical Operator : Logic  Operator=NOT  AllPortsSameDT=off  OutDataTypeStr=boolean
  Pipeline : Delay  InitialCondition=0
  Pipeline1 : Delay  InitialCondition=0
  Pipeline2 : Delay  DelayLength=1  InitialCondition=0
  Pipeline3 : Delay  DelayLength=1  InitialCondition=0
  Pipeline4 : Delay  DelayLength=1  InitialCondition=0
  Preamble Address Counter : hdlsllib/Sources/HDL Counter  CountType=Count limited  CountInit=0  CountStep=1  CountMax=128  CountFromType=Initial value  CountFrom=0  CountResetPort=on  CountLoadPort=off  CountEnbPort=on  CountDirPort=off  CountHitOutputPort=off  CountDataType=Unsigned  CountWordLen=16  CountFracLen=0  CountSampTime=1
  Preamble Data Mux : Switch  Criteria=u2 ~= 0  SaturateOnIntegerOverflow=off  InputSameDT=off
  data lookup : LookupNDDirect  NumberOfTableDimensions=1  Table=qam_params.tx_data_bits  DiagnosticForOutOfRangeInput=Error  SampleTime=1/qam_params.bitRate  TableDataTypeStr=boolean
  preamble lookup : LookupNDDirect  NumberOfTableDimensions=1  Table=qam_params.preamble_bits  DiagnosticForOutOfRangeInput=Error  SampleTime=1/qam_params.bitRate  TableDataTypeStr=boolean
  packet_bits : Outport  VectorParamsAs1DForOutWhenUnconnected=off
  wires:
  Logical Operator/1 -> Pipeline1/1
  load preamble/1 -> Preamble Address Counter/2
  load data/1 -> Pipeline2/1, Logical Operator/1, Data Address Counter/1
  Preamble Data Mux/1 -> packet_bits/1
  Pipeline1/1 -> Preamble Data Mux/2
  Pipeline/1 -> Preamble Data Mux/1
  Pipeline4/1 -> Preamble Data Mux/3
  preamble lookup/1 -> Pipeline/1
  Pipeline3/1 -> HDL Data Scrambler/1(Data_In)
  data lookup/1 -> Pipeline3/1
  Data Address Counter/1 -> data lookup/1
  Pipeline2/1 -> HDL Data Scrambler/Enable
  HDL Data Scrambler/1(Scrambled_Out) -> Pipeline4/1
  Preamble Address Counter/1 -> preamble lookup/1
  reset preamble/1 -> Preamble Address Counter/1

== system comm8qamtxrxhdl/QAM Tx HDL/Data Generation & Packetization/Group Bits ==
  Bits In : Inport
  Bit Concat : hdlsllib/Logic and Bit Operations/Bit Concat  numInputs=3
  Delay4 : Delay  InitialCondition=0
  Delay5 : Delay  DelayLength=1  InitialCondition=0
  Downsample : DownSample  N=3  phase=2  RateOptions=Allow multirate processing
  Integer Out : Outport  VectorParamsAs1DForOutWhenUnconnected=off
  wires:
  Bits In/1 -> Delay4/1, Delay5/1, Bit Concat/3
  Delay4/1 -> Bit Concat/1
  Delay5/1 -> Bit Concat/2
  Bit Concat/1 -> Downsample/1
  Downsample/1 -> Integer Out/1

== system comm8qamtxrxhdl/QAM Rx HDL/Coarse Frequency Offset Correction/Frequency Offset Estimation/Enabled Wire ==
  In1 : Inport
  Enable : EnablePort
  Out1 : Outport  InitialOutput=0  VectorParamsAs1DForOutWhenUnconnected=off
  wires:
  In1/1 -> Out1/1

== system comm8qamtxrxhdl/QAM Rx HDL/Coarse Frequency Offset Correction/Frequency Offset Estimation/Raise to Power 4 ==
  In1 : Inport
  Delay1 : Delay  InitialCondition=0
  Delay4 : Delay  DelayLength=4  InitialCondition=0
  Delay5 : Delay  DelayLength=4  InitialCondition=0
  Product : Product  OutDataTypeStr=fixdt(1,16,15)
  Product1 : Product  OutDataTypeStr=fixdt(1,16,15)
  Out1 : Outport  VectorParamsAs1DForOutWhenUnconnected=off
  wires:
  Product/1 -> Delay4/1
  Product1/1 -> Delay5/1
  Delay5/1 -> Out1/1
  Delay4/1 -> Product1/2, Product1/1
  In1/1 -> Delay1/1
  Delay1/1 -> Product/2, Product/1

== system comm8qamtxrxhdl/QAM Tx HDL/Data Generation & Packetization/Data Source/HDL Data Scrambler ==
  note: HDL optimized scrambler, implementing the scrambler polynomial [1 1 1 0 1],
      |  with initial states [0 0 0 0]
  Data_In : Inport
  Enable : EnablePort
  BIT_XOR : Logic  Operator=XOR  IconShape=distinctive  AllPortsSameDT=off  OutDataTypeStr=boolean
  BIT_XOR1 : Logic  Operator=XOR  IconShape=distinctive  AllPortsSameDT=off  OutDataTypeStr=boolean
  BIT_XOR2 : Logic  Operator=XOR  IconShape=distinctive  AllPortsSameDT=off  OutDataTypeStr=boolean
  p{1..4} (4 alike) : Delay  DelayLength=1
  Scrambled_Out : Outport  InitialOutput=0  VectorParamsAs1DForOutWhenUnconnected=off
  wires:
  BIT_XOR2/1 -> Scrambled_Out/1, p1/1
  p4/1 -> BIT_XOR/2
  p1/1 -> p2/1, BIT_XOR1/1
  BIT_XOR/1 -> BIT_XOR1/2
  p3/1 -> p4/1
  p2/1 -> BIT_XOR/1, p3/1
  BIT_XOR1/1 -> BIT_XOR2/2
  Data_In/1 -> BIT_XOR2/1

== matlab function comm8qamtxrxhdl/QAM Rx HDL/Timing Recovery/Interpolation Control ==
  data: Delta input; Underflow output; mu output
function [Underflow, mu] = Interpolation_ctrl(Delta)
% Implementation of modulo-1 counter for interpolation control listed in
% Figure 8.4.19 of "Digital Communications - A Discrete-Time Approach"
% by Michael Rice. See design details in Chapter 8.4.3 of the same book.
% 
% Input:
%   Delta - Loop filter output. If loop is in lock, delta would be small
% Output:
%   Underflow - Indicator of counter underflow. This is the strobe signal
%               for downstream processing
%   mu - Difference between actual sampling instant and the optimal instant,
%        between zero and one
%#codegen

% delay1 - Counter value delayed by 1 sample
% Regtemp - The estimated timing error normalized by half QPSK symbols

W = 16; % accumulator wordlength
F = 15; % accumulator fraction length

persistent delay1 Regtemp;  
if isempty(delay1)
    delay1  = fi(0,1,W,F);
    Regtemp = fi(0,1,W,F);
end

mask = fi(1-2^(-F),1,W,F);

counter = bitand(mask,delay1)-Delta-fi(0.5,1,W,F); % decrementing counter
% if delay1 is a nonnegative number,
% then mod(delay1,1) equals the fractional part of delay1

if counter < 0
    Underflow = true;
    Regtemp = bitshift(bitand(mask,delay1),1);     
else
    Underflow = false;
end

mu = Regtemp;

% Update delay buffer
% delay1 = counter;
if counter<0
    delay1 = fi(counter+1,1,W,F); %make sure delay1 is nonnegative
else
    delay1 = fi(counter,1,W,F);
end

== matlab function comm8qamtxrxhdl/QAM Rx HDL/Timing Recovery/Timing Error Detector ==
  data: In input; strobe input; e output
function e = TED(In, strobe)
% Zero-Crossing Timing Error Detector. See "Zero-Crossing Timing Error
% Detector" section in Chapter 8.4.1 of "Digital Communications - A
% Discrete-Time Approach" by Michael Rice. For bit stuffing/stripping
% details, see page 490-494 of the same book.
%
% Input: 
%   In - Input samples, interpolation result
%   strobe - Signal to enable timing error calculation
% Output:
%   e - Timing error
%#codegen

persistent delay1_R delay1_I delay2_R delay2_I delayStrobe; 
% Input delayed by one and 2 samples, and
% Enable signal delayed by one sample
if isempty(delay1_R)    
    delay1_R=fi(0,1,16,15);
    delay1_I=fi(0,1,16,15);
    delay2_R=fi(0,1,16,15);
    delay2_I=fi(0,1,16,15);    
    delayStrobe = false;
end

In_Real = real(In);
In_Imag = imag(In);

if strobe==true && delayStrobe~=strobe
    if ( bitget(delay2_R,16)==bitget(In_Real,16) )         
        OP1=fi(0,1,16,15);
    elseif bitget(delay2_R,16)==true         
        OP1=fi(-1*bitshift(delay1_R,1),1,16,15);
    else        
        OP1=fi(bitshift(delay1_R,1),1,16,15);
    end
    
    if ( bitget(delay2_I,16)==bitget(In_Imag,16) )        
        OP2=fi(0,1,16,15);
    elseif bitget(delay2_I,16)==true        
        OP2=fi(-1*bitshift(delay1_I,1),1,16,15);
    else        
        OP2=fi(bitshift(delay1_I,1),1,16,15);
    end
else
    OP1=fi(0,1,16,15);
    OP2=fi(0,1,16,15);
end

e = fi(OP1+OP2,1,16,15);


if delayStrobe~=strobe
    % Shift contents in delay register
    delay2_R = delay1_R;
    delay1_R = In_Real;
    delay2_I = delay1_I;
    delay1_I = In_Imag;
elseif strobe==true
    % Two consecutive high strobes
    delay2_R = fi(0,1,16,15); % Stuff missing sample
    delay1_R = In_Real; 
    delay2_I = fi(0,1,16,15); % Stuff missing sample
    delay1_I = In_Imag; 
end

% If both current and previous enable signals are 0, skip current sample
% and keep the delayed signals unchanged. (Bit stripping)
delayStrobe = strobe;

== matlab function comm8qamtxrxhdl/QAM Rx HDL/Demodulate/Rectangular QAM Demodulator Baseband ==
  data: u input; y output
function y = Rect8QAMDemod(u)
%#codegen
% HDL-compatible Gray-coded 8-QAM Hard-Decision Demodulator (MinDist = 2)
% Constellation points: I in {-3, -1, +1, +3}, Q in {-1, +1}
I = real(u);
Q = imag(u);
b1 = (I >= 0);       % MSB: 0 for I < 0, 1 for I >= 0
b2 = (abs(I) <= 2);  % Mid: 0 for |I| > 2 (+-3), 1 for |I| <= 2 (+-1)
b3 = (Q < 0);        % LSB: 0 for Q >= 0 (+1), 1 for Q < 0 (-1)
y  = [b1; b2; b3];

== matlab function comm8qamtxrxhdl/QAM Tx HDL/Data Generation & Packetization/Controller FSM ==
  data: reset_preamble output; load_preamble output; load_data output
function [reset_preamble,load_preamble, load_data] = ControllerFSM()
%#codegen

persistent packState;
persistent stateCounter;

sType = numerictype(0,1,0);
cType = numerictype(0,8,0);

if isempty(packState)
    packState = fi(0,'numerictype',sType);
    stateCounter  = fi(0,'numerictype',cType);
end

Pack_Preamble = fi(0,'numerictype',sType);
Append_Data   = fi(1,'numerictype',sType);

switch(packState)
    case Pack_Preamble  %% Pack_Preamble
        load_preamble  = true;
        reset_preamble = false;
        load_data      = false;
        
        if stateCounter == 41;  %% Pack_Preamble complete
            packState(:) = 1;                   %% move to Append_Data state
            stateCounter(:) = 0;                %% reset counter
        else
            packState(:) = 0;                   %% remain in Pack_Preamble state
            stateCounter(:) = stateCounter +1;  %% increment preamble count
        end
        
    case Append_Data    %% Append_Data
        load_preamble  = false;
        reset_preamble = true;
        load_data      = true;
        
        if stateCounter == 125  %% Append_Data complete
            packState(:) = 0;                   %% move to Pack_Preamble state
            stateCounter(:) = 0;                %% reset counter
        else
            packState(:) = 1;                   %% remain in Append_Data state
            stateCounter(:) = stateCounter +1;  %% increment data count
        end
        
    otherwise
        load_preamble  = false;
        reset_preamble = false;
        load_data      = false;
        stateCounter(:) = 0;
end

== matlab function comm8qamtxrxhdl/Text Message Decoding/  ==
  data: newPacket input; dValid input; RxGo output; framed_data output; bit1 input; bit2 input; bit3 input
function [RxGo,framed_data] = dataframer(newPacket, dValid, bit1, bit2, bit3)
%#codegen

persistent gooddata_so_far frame_index

if isempty(gooddata_so_far)
    gooddata_so_far = false(168,1);
    frame_index = 1;
end

RxGo = false;
framed_data = false(168,1);

if dValid==true
    gooddata_so_far(frame_index:frame_index+2) = [bit1 bit2 bit3];
    frame_index = frame_index+3;
    if (frame_index==169) || (newPacket==true)
        RxGo = true;
        framed_data = gooddata_so_far;
        frame_index = 1;
    end
end

== matlab function comm8qamtxrxhdl/QAM Rx HDL/Magnitude & Phase Recovery/MATLAB Function3 ==
  data: dvalid output; enable input; isPreamble output
function [dvalid,isPreamble] = fcn(enable)
%#codegen

persistent state;
persistent counter;


if isempty(state);
    state      = false;
    counter    = uint8(0);
end


if counter > 42
    isPreamble = true;
else
    isPreamble = false;
end


if state==false
    dvalid=false;
else %state==true
    dvalid=true;
    counter = counter-1;
end


% state transition
if state==false && enable==true
    state=true;
    counter=uint8(56);
elseif state==true && counter==0
    if enable==true % packages come back-to-back
        state      = true;
        counter    = uint8(56);
    else
        state = false;    
    end
end

== matlab function comm8qamtxrxhdl/Text Message Decoding/Descramble and Print/BitsToDecimal1 ==
  data: u input
function BitsToASCII(u)
% Convert bits to ASCII message (8-QAM Option A: 18 chars = 126 bits).

persistent package_counter;
persistent error_counter;
if isempty(package_counter)
    package_counter = 0;
    error_counter   = 0;
end

coder.extrinsic('disp')
coder.extrinsic('num2str')

aa = de2bi(int8('Hello! ~8-QAM~ 0'),7,'left-msb');
bits_ref = double(reshape(aa.',1,[]));
bits_ref = bits_ref(:);

error_counter   = error_counter   + sum(abs(bits_ref - u(1:112)));
package_counter = package_counter + 1;

% Convert binary-valued column vector to 7-bit decimal values.
w = [64 32 16 8 4 2 1]; % binary digit weighting
Nbits = numel(u);
Ny = Nbits/7;
y = zeros(1,Ny);
for i = 0:Ny-1
    y(i+1) = w*u(7*i+(1:7));
end

% Display ASCII message to command window
if rem(package_counter,50)==0
    disp([char(y) '    ==>    BER = ' num2str(error_counter/50/7/16)]);
    error_counter = 0;
else
    disp(char(y));
end
